simulink model "test_SimulinkMdl2_Baseline"  (R2021b)
settings: Solver=FixedStepAuto  StartTime=0.0  StopTime=OutTable.Time(end)  FixedStep=DT  RelTol=1e-3
values from neighbouring files (symbols this model uses):
  DT = 0.008    [LUTMFile.m]    (also in UIOLinestTr.m; exUIO_WECS.m; getFictInputMatricesOrd3M.m; initWorkspace.m)
  Lin_points = 0.74811652133345019 0.78122947334555715 0.82586806925039735 0.88042797952230989 0.94564154658981237 1.06231329175348 1.1780905557148451 1.2402773842094346 1.254474305465946 1.2544764615597244 1.2544775037226534 1.2544778841663968 1.2544780221694662 1.2544779823335293 1.254477987181289 1.2544781738200332 1.254478189259095 1.2544780953600987 1.2544781548505395 1.2544783366942183 1.2544785605869417 1    [DD_test.sldd]    (also in LinPointsMFile.m = struct)
undefined symbols (not defined in the file or in its folder): Rotor_Lambda
settings Model: DataDictionary=DD_test.sldd  Creator=Hazim Namik  LastModifiedBy=ditt_aj
settings SolverCC: AlgebraicLoopSolver=TrustRegion
settings DataIOCC: LimitDataPoints=on  SaveFormat=Array  ReturnWorkspaceOutputs=off
settings OptimizationCC: BlockReduction=off  BooleanDataType=off  LifeSpan=inf
settings DebuggingCC: SaveWithParameterizedLinksMsg=none  UnderspecifiedInitializationDetection=Classic  MergeDetectMultiDrivingBlocksExec=none  SignalResolutionControl=TryResolveAllWithWarning  SFUnexpectedBacktrackingDiag=warning  SFNoUnconditionalDefaultTransitionDiag=warning  SFExecutionAtInitializationDiag=none  SFMachineParentedDataDiag=warning  ArithmeticOperatorsInVariantConditions=warning
settings HardwareCC: ProdBitPerPointer=32  ProdBitPerSizeT=32  ProdBitPerPtrDiffT=32  ProdLargestAtomicFloat=None  ProdIntDivRoundTo=Undefined  ProdEndianess=Unspecified  ProdWordSize=32  ProdHWDeviceType=32-bit Generic  TargetUnknown=on
settings ModelReferenceCC: PropagateSignalLabelsOutOfModel=off
settings SFSimCC: SimUseLocalCustomCode=off  CustomCodeUndefinedFunction=UseInterfaceOnly
settings RTWCC: RTWUseLocalCustomCode=off
settings CodeAppCC: StateflowObjectComments=on
settings GRTTargetCC: TargetLangStandard=C89/C90 (ANSI)
settings ConfigComp: CovMetricSettings=dw  CovSaveCumulativeToWorkspaceVar=on  CovSaveSingleToWorkspaceVar=on  CovExternalEMLEnable=off

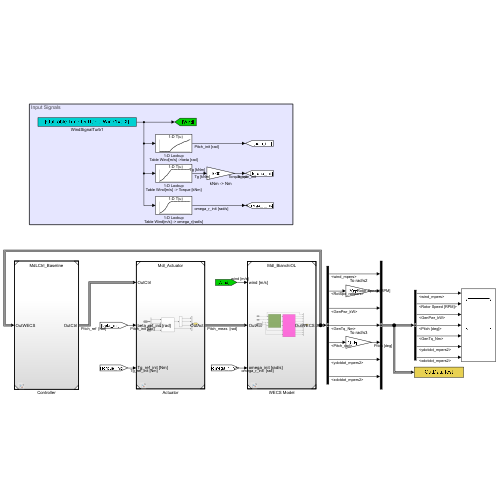
[thumbnail: Simulink's stored preview of the top-level diagram]
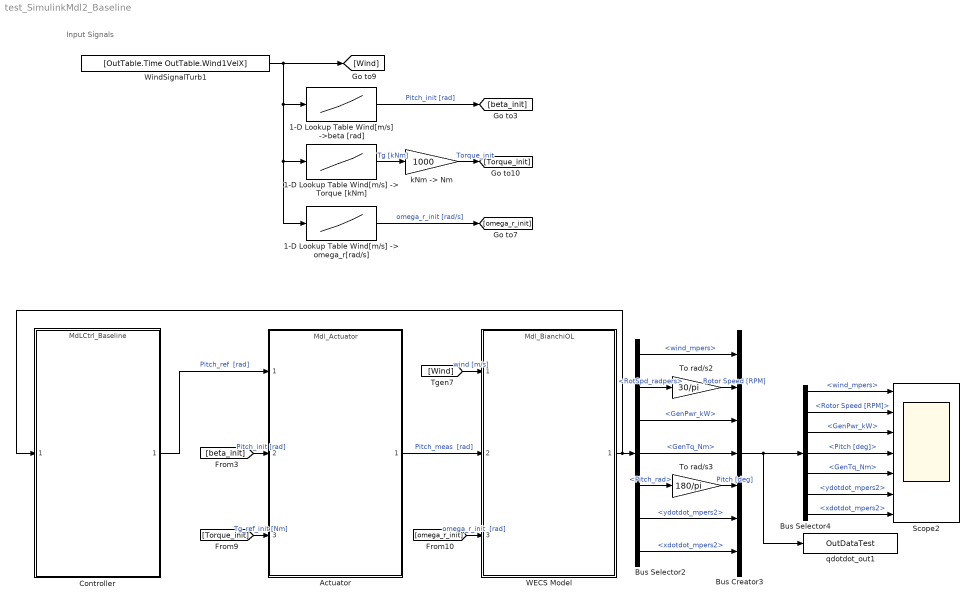
== system test_SimulinkMdl2_Baseline ==
  note: Input Signals
  "1-D Lookup Table Wind[m/s] -> Torque [kNm]" : Lookup_n-D  NumberOfTableDimensions=1  BreakpointsForDimension1=Lin_points.V  BreakpointsForDimension2=Rotor_Lambda  Table=Lin_points.Torque  InternalRulePriority=Speed  RndMeth=Simplest  InputSameDT=on
  "1-D Lookup Table Wind[m/s] -> omega_r[rad/s]" : Lookup_n-D  NumberOfTableDimensions=1  BreakpointsForDimension1=Lin_points.V  BreakpointsForDimension2=Rotor_Lambda  Table=Lin_points.RSpeed  InternalRulePriority=Speed  RndMeth=Simplest  InputSameDT=on
  1-D Lookup Table Wind[m/s] ->beta [rad] : Lookup_n-D  NumberOfTableDimensions=1  BreakpointsForDimension1=Lin_points.V  BreakpointsForDimension2=Rotor_Lambda  Table=Lin_points.Pitch  InternalRulePriority=Speed  RndMeth=Simplest  InputSameDT=on
  Actuator : ModelReference  ModelNameDialog=Mdl_Actuator.slx  SimulationMode=Normal  ModelReferenceVersion=4.0
  Bus Creator3 : BusCreator  Inputs=7
  Bus Selector2 : BusSelector  OutputSignals=wind_mpers,RotSpd_radpers,GenPwr_kW,GenTq_Nm,Pitch_rad,ydotdot_mpers2,xdotdot_mpers2
  Bus Selector4 : BusSelector  OutputSignals=wind_mpers,Rotor Speed [RPM],GenPwr_kW,Pitch [deg],GenTq_Nm,ydotdot_mpers2,xdotdot_mpers2
  Controller : ModelReference  ModelNameDialog=MdLCtrl_Baseline.slx  SimulationMode=Normal  ModelReferenceVersion=1.24
  Scope2 : Scope  NumInputPorts=7
      settings: Tag=Scope
  To rad/s2 : Gain  Gain=30/pi
  To rad/s3 : Gain  Gain=180/pi
  WECS Model : ModelReference  ModelNameDialog=Mdl_BianchiOL.slx  SimulationMode=Normal  ModelReferenceVersion=4.9
  WindSignalTurb1 : FromWorkspace  VariableName=[OutTable.Time OutTable.Wind1VelX]  SampleTime=DT  OutputAfterFinalValue=Holding final value
  "kNm -> Nm" : Gain  Gain=1000
  qdotdot_out1 : ToWorkspace  VariableName=OutDataTest  SampleTime=-1
  wires:
  [Torque_init] -> Actuator/3  "Tg_ref_init [Nm]"
  "1-D Lookup Table Wind[m/s] -> Torque [kNm]"/1 -> "kNm -> Nm"/1  "Tg [kNm]"
  "1-D Lookup Table Wind[m/s] -> omega_r[rad/s]"/1 -> [omega_r_init]  "omega_r_init [rad/s]"
  Actuator/1 -> WECS Model/2  "Pitch_meas  [rad]"
  [Wind] -> WECS Model/1  "wind [m/s]"
  WindSignalTurb1/1 -> [Wind], "1-D Lookup Table Wind[m/s] -> omega_r[rad/s]"/1, "1-D Lookup Table Wind[m/s] -> Torque [kNm]"/1, 1-D Lookup Table Wind[m/s] ->beta [rad]/1
  "kNm -> Nm"/1 -> [Torque_init]  "Torque_init"
  1-D Lookup Table Wind[m/s] ->beta [rad]/1 -> [beta_init]  "Pitch_init [rad]"
  [omega_r_init] -> WECS Model/3  "omega_r_init  [rad]"
  Controller/1 -> Actuator/1  "Pitch_ref  [rad]"
  [beta_init] -> Actuator/2  "Pitch_init [rad]"
  Bus Selector4/5 -> Scope2/5  "<GenTq_Nm>"
  To rad/s3/1 -> Bus Creator3/5  "Pitch [deg]"
  Bus Selector4/1 -> Scope2/1  "<wind_mpers>"
  Bus Selector4/7 -> Scope2/7  "<xdotdot_mpers2>"
  Bus Selector4/6 -> Scope2/6  "<ydotdot_mpers2>"
  Bus Creator3/1 -> Bus Selector4/1, qdotdot_out1/1
  Bus Selector4/4 -> Scope2/4  "<Pitch [deg]>"
  To rad/s2/1 -> Bus Creator3/2  "Rotor Speed [RPM]"
  Bus Selector2/7 -> Bus Creator3/7  "<xdotdot_mpers2>"
  Bus Selector2/6 -> Bus Creator3/6  "<ydotdot_mpers2>"
  Bus Selector2/5 -> To rad/s3/1  "<Pitch_rad>"
  Bus Selector4/3 -> Scope2/3  "<GenPwr_kW>"
  Bus Selector4/2 -> Scope2/2  "<Rotor Speed [RPM]>"
  Bus Selector2/1 -> Bus Creator3/1  "<wind_mpers>"
  Bus Selector2/3 -> Bus Creator3/3  "<GenPwr_kW>"
  Bus Selector2/4 -> Bus Creator3/4  "<GenTq_Nm>"
  Bus Selector2/2 -> To rad/s2/1  "<RotSpd_radpers>"
  WECS Model/1 -> Controller/1, Bus Selector2/1
